simulink subsystem "oswec_translational_pto"  (R2025b)
settings: Solver=VariableStepAuto  StartTime=0.0  StopTime=10.0  RelTol=1e-3
undefined symbols (not defined in the file or in its folder): body, constraint, pto
libraries: WECSim_Lib_Constraints x4, WECSim_Lib_Body_Elements x2, WECSim_Lib_Frames x1, sm_lib x1, WECSim_Lib_PTOs x1
settings Model: Creator=ndegoede  LastModifiedBy=ndegoede

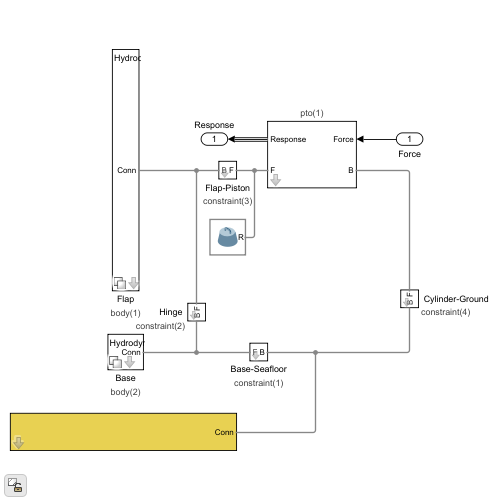
[thumbnail: Simulink's stored preview of the top-level diagram]
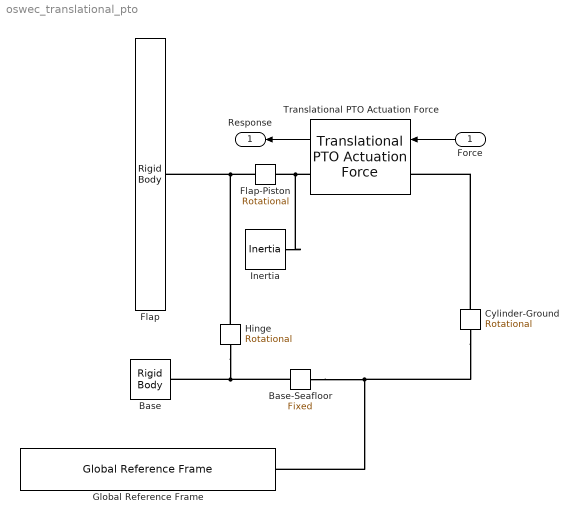
== system oswec_translational_pto ==
  Force : Inport
  Base : WECSim_Lib_Body_Elements/Rigid Body  body=body(2)
  Base-Seafloor : WECSim_Lib_Constraints/Fixed  constraint=constraint(1)
      settings: AttributesFormatString=%<constraint>
  Cylinder-Ground : WECSim_Lib_Constraints/Rotational  constraint=constraint(4)
      settings: AttributesFormatString=%<constraint>
  Flap : WECSim_Lib_Body_Elements/Rigid Body  body=body(1)
  Flap-Piston : WECSim_Lib_Constraints/Rotational  constraint=constraint(3)
      settings: AttributesFormatString=%<constraint>
  Global Reference Frame : WECSim_Lib_Frames/Global Reference Frame  waves=waves  simu=simu
  Hinge : WECSim_Lib_Constraints/Rotational  constraint=constraint(2)
      settings: AttributesFormatString=%<constraint>
  Inertia : sm_lib/Body Elements/Inertia  InertiaType=PointMass  Mass=1  MassUnits=kg  CenterOfMass=[0 0 0]  CenterOfMassUnits=m  MomentsOfInertia=[1 1 1]  MomentsOfInertiaUnits=kg*m^2  ProductsOfInertia=[0 0 0]  ProductsOfInertiaUnits=kg*m^2  GraphicType=Marker  MarkerShape=Inertia  MarkerSize=20  GraphicVisPropType=SimpleVisualProperties  GraphicDiffuseColor=[0.5 0.5 0.5]  GraphicOpacity=1  GraphicSpecularColor=[0.5 0.5 0.5 1.0]  GraphicAmbientColor=[0.15 0.15 0.15 1.0]  GraphicEmissiveColor=[0.0 0.0 0.0 1.0]  GraphicShininess=75
  Translational PTO Actuation Force : WECSim_Lib_PTOs/Translational PTO Actuation Force  pto=pto(1)
      settings: AttributesFormatString=%<pto>
  Response : Outport
  wires:
  Force/1 -> Translational PTO Actuation Force/1
  Translational PTO Actuation Force/1 -> Response/1
  connections:
  Flap-Piston/LConn1 -- Flap/RConn1 -- Hinge/RConn1
  Cylinder-Ground/LConn1 -- Global Reference Frame/RConn1 -- Base-Seafloor/LConn1
  Base-Seafloor/RConn1 -- Base/RConn1 -- Hinge/LConn1
  Cylinder-Ground/RConn1 -- Translational PTO Actuation Force/LConn1
  Translational PTO Actuation Force/RConn1 -- Inertia/RConn1 -- Flap-Piston/RConn1
